simulink model "azimuth_wiith_variable_gain"  (R2025b)
settings: Solver=VariableStepAuto  StartTime=0.0  StopTime=10.0  RelTol=1e-3
values from neighbouring files (symbols this model uses):
  Kfar = 300    [nl_gain_demo.m]    (also in pVsScheduledPd.m)
  Knear = 60    [nl_gain_demo.m]    (also in pVsScheduledPd.m)
libraries: fl_lib x86, nesl_utility x15, simulink x2
settings Model: Creator=Lenovo  LastModifiedBy=Lenovo

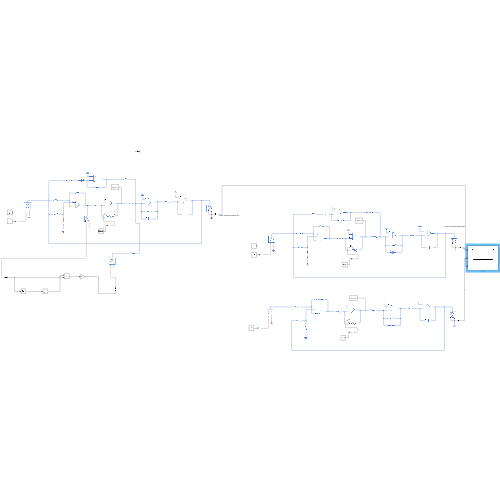
[thumbnail: Simulink's stored preview of the top-level diagram]
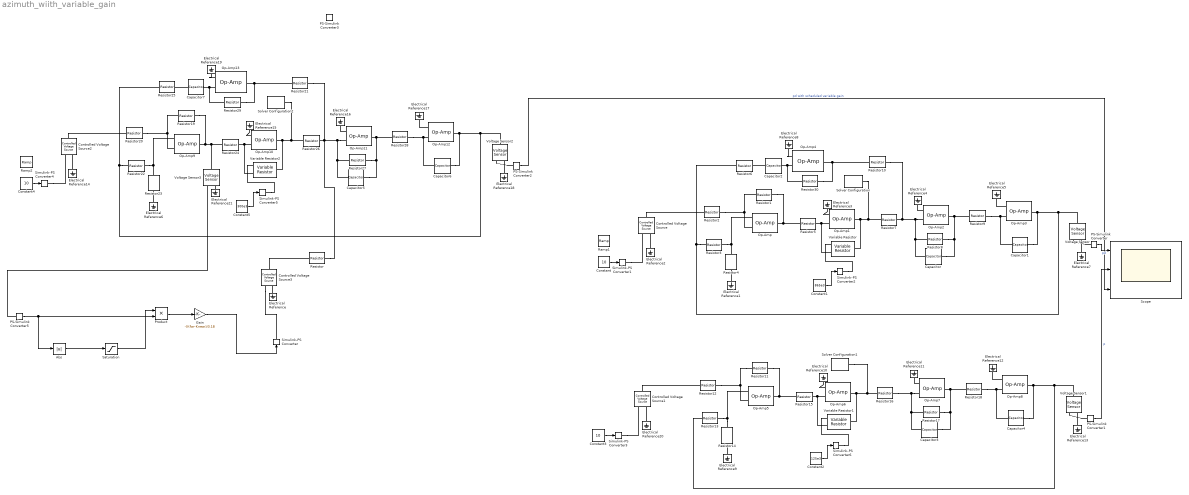
== system azimuth_wiith_variable_gain ==
  Abs : Abs  SaturateOnIntegerOverflow=off
  Capacitor{,1..7} (8 alike) : fl_lib/Electrical/Electrical Elements/Capacitor  c=1e-6 F  r=1e-6 Ohm  g=0 1/Ohm  i_specify=off  i_priority=None  i=0 A  i_nominal_specify=off  i_nominal_value=1  i_nominal_unit=A  v_specify=off  v_priority=None  v=0 V  v_nominal_specify=off  v_nominal_value=1  v_nominal_unit=V  vc_specify=off  vc_priority=High  vc=0 V  vc_nominal_specify=off  vc_nominal_value=1  vc_nominal_unit=V
  Constant : Constant  Value=10
  Constant1 : Constant  Value=865e3
  Constant2 : Constant  Value=125e3
  Constant3 : Constant  Value=10
  Constant4 : Constant  Value=10
  Constant5 : Constant  Value=300e3
  Controlled Voltage Source{,1..3} (4 alike) : fl_lib/Electrical/Electrical Sources/Controlled Voltage Source
  Electrical Reference{,1..21} (22 alike) : fl_lib/Electrical/Electrical Elements/Electrical Reference
  Gain : Gain  Gain=-(Kfar-Knear)/3.18
  Op-Amp{,1..13} (14 alike) : fl_lib/Electrical/Electrical Elements/Op-Amp  outI_specify=off  outI_priority=None  outI=0 A  outI_nominal_specify=off  outI_nominal_value=1  outI_nominal_unit=A
  PS-Simulink Converter{,1..3,5} (5 alike) : nesl_utility/PS-Simulink Converter  PhysicalDomain=network_engine_domain  SubClassName=ps_output  LeftPortType=input  RightPortType=output  PseudoPeriodic=off  Frequencies=[]  VectorFormat=inherit  Unit=inherit  AffineConversion=off
  Product : Product
  Ramp1 : simulink/Sources/Ramp  slope=1  start=0  InitialOutput=0
  Ramp2 : simulink/Sources/Ramp  slope=1  start=0  InitialOutput=0
  Resistor : fl_lib/Electrical/Electrical Elements/Resistor  R=4.87 MOhm  i_specify=off  i_priority=None  i=0 A  i_nominal_specify=off  i_nominal_value=1  i_nominal_unit=A  v_specify=off  v_priority=None  v=0 V  v_nominal_specify=off  v_nominal_value=1  v_nominal_unit=V
  Resistor{1,4,11,14,19,23} (6 alike) : fl_lib/Electrical/Electrical Elements/Resistor  R=31.8 kOhm  i_specify=off  i_priority=None  i=0 A  i_nominal_specify=off  i_nominal_value=1  i_nominal_unit=A  v_specify=off  v_priority=None  v=0 V  v_nominal_specify=off  v_nominal_value=1  v_nominal_unit=V
  Resistor10 : fl_lib/Electrical/Electrical Elements/Resistor  R=4.87 MOhm  i_specify=off  i_priority=None  i=0 A  i_nominal_specify=off  i_nominal_value=1  i_nominal_unit=A  v_specify=off  v_priority=None  v=0 V  v_nominal_specify=off  v_nominal_value=1  v_nominal_unit=V
  Resistor{2..3,12..13,20,22} (6 alike) : fl_lib/Electrical/Electrical Elements/Resistor  R=100 kOhm  i_specify=off  i_priority=None  i=0 A  i_nominal_specify=off  i_nominal_value=1  i_nominal_unit=A  v_specify=off  v_priority=None  v=0 V  v_nominal_specify=off  v_nominal_value=1  v_nominal_unit=V
  Resistor15 : fl_lib/Electrical/Electrical Elements/Resistor  R=5 kOhm  i_specify=off  i_priority=None  i=0 A  i_nominal_specify=off  i_nominal_value=1  i_nominal_unit=A  v_specify=off  v_priority=None  v=0 V  v_nominal_specify=off  v_nominal_value=1  v_nominal_unit=V
  Resistor16 : fl_lib/Electrical/Electrical Elements/Resistor  R=4.8 MOhm  i_specify=off  i_priority=None  i=0 A  i_nominal_specify=off  i_nominal_value=1  i_nominal_unit=A  v_specify=off  v_priority=None  v=0 V  v_nominal_specify=off  v_nominal_value=1  v_nominal_unit=V
  Resistor17 : fl_lib/Electrical/Electrical Elements/Resistor  R=585 kOhm  i_specify=off  i_priority=None  i=0 A  i_nominal_specify=off  i_nominal_value=1  i_nominal_unit=A  v_specify=off  v_priority=None  v=0 V  v_nominal_specify=off  v_nominal_value=1  v_nominal_unit=V
  Resistor18 : fl_lib/Electrical/Electrical Elements/Resistor  R=1 MOhm  i_specify=off  i_priority=None  i=0 A  i_nominal_specify=off  i_nominal_value=1  i_nominal_unit=A  v_specify=off  v_priority=None  v=0 V  v_nominal_specify=off  v_nominal_value=1  v_nominal_unit=V
  Resistor21 : fl_lib/Electrical/Electrical Elements/Resistor  R=4.87 MOhm  i_specify=off  i_priority=None  i=0 A  i_nominal_specify=off  i_nominal_value=1  i_nominal_unit=A  v_specify=off  v_priority=None  v=0 V  v_nominal_specify=off  v_nominal_value=1  v_nominal_unit=V
  Resistor24 : fl_lib/Electrical/Electrical Elements/Resistor  R=5 kOhm  i_specify=off  i_priority=None  i=0 A  i_nominal_specify=off  i_nominal_value=1  i_nominal_unit=A  v_specify=off  v_priority=None  v=0 V  v_nominal_specify=off  v_nominal_value=1  v_nominal_unit=V
  Resistor25 : fl_lib/Electrical/Electrical Elements/Resistor  R=10 kOhm  i_specify=off  i_priority=None  i=0 A  i_nominal_specify=off  i_nominal_value=1  i_nominal_unit=A  v_specify=off  v_priority=None  v=0 V  v_nominal_specify=off  v_nominal_value=1  v_nominal_unit=V
  Resistor26 : fl_lib/Electrical/Electrical Elements/Resistor  R=4.8 MOhm  i_specify=off  i_priority=None  i=0 A  i_nominal_specify=off  i_nominal_value=1  i_nominal_unit=A  v_specify=off  v_priority=None  v=0 V  v_nominal_specify=off  v_nominal_value=1  v_nominal_unit=V
  Resistor27 : fl_lib/Electrical/Electrical Elements/Resistor  R=585 kOhm  i_specify=off  i_priority=None  i=0 A  i_nominal_specify=off  i_nominal_value=1  i_nominal_unit=A  v_specify=off  v_priority=None  v=0 V  v_nominal_specify=off  v_nominal_value=1  v_nominal_unit=V
  Resistor28 : fl_lib/Electrical/Electrical Elements/Resistor  R=1 MOhm  i_specify=off  i_priority=None  i=0 A  i_nominal_specify=off  i_nominal_value=1  i_nominal_unit=A  v_specify=off  v_priority=None  v=0 V  v_nominal_specify=off  v_nominal_value=1  v_nominal_unit=V
  Resistor29 : fl_lib/Electrical/Electrical Elements/Resistor  R=15 MOhm  i_specify=off  i_priority=None  i=0 A  i_nominal_specify=off  i_nominal_value=1  i_nominal_unit=A  v_specify=off  v_priority=None  v=0 V  v_nominal_specify=off  v_nominal_value=1  v_nominal_unit=V
  Resistor30 : fl_lib/Electrical/Electrical Elements/Resistor  R=11 MOhm  i_specify=off  i_priority=None  i=0 A  i_nominal_specify=off  i_nominal_value=1  i_nominal_unit=A  v_specify=off  v_priority=None  v=0 V  v_nominal_specify=off  v_nominal_value=1  v_nominal_unit=V
  Resistor5 : fl_lib/Electrical/Electrical Elements/Resistor  R=5 kOhm  i_specify=off  i_priority=None  i=0 A  i_nominal_specify=off  i_nominal_value=1  i_nominal_unit=A  v_specify=off  v_priority=None  v=0 V  v_nominal_specify=off  v_nominal_value=1  v_nominal_unit=V
  Resistor6 : fl_lib/Electrical/Electrical Elements/Resistor  R=10 kOhm  i_specify=off  i_priority=None  i=0 A  i_nominal_specify=off  i_nominal_value=1  i_nominal_unit=A  v_specify=off  v_priority=None  v=0 V  v_nominal_specify=off  v_nominal_value=1  v_nominal_unit=V
  Resistor7 : fl_lib/Electrical/Electrical Elements/Resistor  R=4.8 MOhm  i_specify=off  i_priority=None  i=0 A  i_nominal_specify=off  i_nominal_value=1  i_nominal_unit=A  v_specify=off  v_priority=None  v=0 V  v_nominal_specify=off  v_nominal_value=1  v_nominal_unit=V
  Resistor8 : fl_lib/Electrical/Electrical Elements/Resistor  R=585 kOhm  i_specify=off  i_priority=None  i=0 A  i_nominal_specify=off  i_nominal_value=1  i_nominal_unit=A  v_specify=off  v_priority=None  v=0 V  v_nominal_specify=off  v_nominal_value=1  v_nominal_unit=V
  Resistor9 : fl_lib/Electrical/Electrical Elements/Resistor  R=1 MOhm  i_specify=off  i_priority=None  i=0 A  i_nominal_specify=off  i_nominal_value=1  i_nominal_unit=A  v_specify=off  v_priority=None  v=0 V  v_nominal_specify=off  v_nominal_value=1  v_nominal_unit=V
  Saturation : Saturate  UpperLimit=3.18  LowerLimit=0
  Scope : Scope  NumInputPorts=3
      settings: ActiveDisplayYMinimum=-9.3038927314256714  ActiveDisplayYMaximum=26.895222046777043
  Simulink-PS Converter{,1..6} (7 alike) : nesl_utility/Simulink-PS Converter  PhysicalDomain=network_engine_domain  SubClassName=ps_input  LeftPortType=input  RightPortType=output  PseudoPeriodic=off  Frequencies=[]  NoiseDistribution=none  NoiseParameters=[]  Unit=1  AffineConversion=off  FilteringAndDerivatives=provide  SimscapeFilterOrder=1  InputFilterTimeConstant=0.001  UdotUserProvided=0
  Solver Configuration : nesl_utility/Solver Configuration  PhysicalDomain=network_engine_domain  SubClassName=solver  LeftPortType=input  RightPortType=generic  Tones=[]  Harmonics=[]  SimulateNoise=off  Profile=off  UseLocalSampling=off  EnableSwitchedLinearOptims=on  FrequencyDomain=off  UseCCode=off  RelTol=0.001  AbsTol=0.001  MinStep=1e-09  ToWorkspace=off  RevertToSquareIcSolve=off  NumHomotopyIterations=100  PhasorMode=off  PhasorModeNumHarmonics=1  ConsistencySolver=NEWTON_XTOL_AFTER_FTOL  IndexReductionMethod=DerivativeReplacement  DoDC=off  ResidualTolerance=1e-09  ConsistencyTolSource=GLOBAL  ConsistencyAbsTol=0.001  ConsistencyRelTol=0.001  ConsistencyTolFactor=0.001  UseLocalSolver=off  LocalSolverChoice=NE_BACKWARD_EULER_ADVANCER  ResolveIndetEquations=on  FunctionEvalNumThread=1  LocalSolverSampleTime=0.001  DoFixedCost=off  MaxNonlinIter=3  MaxModeIter=2  ComputeImpulses=off  ImpulseIterations=2  LinearAlgebra=auto  LinearAlgebraNumThread=0  EquationFormulation=NE_TIME_EF  DelaysMemoryBudget=1024  AutomaticFiltering=on  FilteringTimeConstant=0.001  PartitionStorageMethod=AS_NEEDED  PartitionMemoryBudget=1024  PartitionMethod=ROBUST  MultibodyUseLocalSolver=off  MultibodyLocalSolverChoice=ODE1  MultibodyLocalSolverSampleTime=0.001
  Solver Configuration1 : nesl_utility/Solver Configuration  PhysicalDomain=network_engine_domain  SubClassName=solver  LeftPortType=input  RightPortType=generic  Tones=[]  Harmonics=[]  SimulateNoise=off  Profile=off  UseLocalSampling=off  EnableSwitchedLinearOptims=on  FrequencyDomain=off  UseCCode=off  RelTol=0.001  AbsTol=0.001  MinStep=1e-09  ToWorkspace=off  RevertToSquareIcSolve=off  NumHomotopyIterations=100  PhasorMode=off  PhasorModeNumHarmonics=1  ConsistencySolver=NEWTON_XTOL_AFTER_FTOL  IndexReductionMethod=DerivativeReplacement  DoDC=off  ResidualTolerance=1e-09  ConsistencyTolSource=GLOBAL  ConsistencyAbsTol=0.001  ConsistencyRelTol=0.001  ConsistencyTolFactor=0.001  UseLocalSolver=off  LocalSolverChoice=NE_BACKWARD_EULER_ADVANCER  ResolveIndetEquations=on  FunctionEvalNumThread=1  LocalSolverSampleTime=0.001  DoFixedCost=off  MaxNonlinIter=3  MaxModeIter=2  ComputeImpulses=off  ImpulseIterations=2  LinearAlgebra=auto  LinearAlgebraNumThread=0  EquationFormulation=NE_TIME_EF  DelaysMemoryBudget=1024  AutomaticFiltering=on  FilteringTimeConstant=0.001  PartitionStorageMethod=AS_NEEDED  PartitionMemoryBudget=1024  PartitionMethod=ROBUST  MultibodyUseLocalSolver=off  MultibodyLocalSolverChoice=ODE1  MultibodyLocalSolverSampleTime=0.001
  Solver Configuration2 : nesl_utility/Solver Configuration  PhysicalDomain=network_engine_domain  SubClassName=solver  LeftPortType=input  RightPortType=generic  Tones=[]  Harmonics=[]  SimulateNoise=off  Profile=off  UseLocalSampling=off  EnableSwitchedLinearOptims=on  FrequencyDomain=off  UseCCode=off  RelTol=0.001  AbsTol=0.001  MinStep=1e-09  ToWorkspace=off  RevertToSquareIcSolve=off  NumHomotopyIterations=100  PhasorMode=off  PhasorModeNumHarmonics=1  ConsistencySolver=NEWTON_XTOL_AFTER_FTOL  IndexReductionMethod=DerivativeReplacement  DoDC=off  ResidualTolerance=1e-09  ConsistencyTolSource=GLOBAL  ConsistencyAbsTol=0.001  ConsistencyRelTol=0.001  ConsistencyTolFactor=0.001  UseLocalSolver=off  LocalSolverChoice=NE_BACKWARD_EULER_ADVANCER  ResolveIndetEquations=on  FunctionEvalNumThread=1  LocalSolverSampleTime=0.001  DoFixedCost=off  MaxNonlinIter=3  MaxModeIter=2  ComputeImpulses=off  ImpulseIterations=2  LinearAlgebra=auto  LinearAlgebraNumThread=0  EquationFormulation=NE_TIME_EF  DelaysMemoryBudget=1024  AutomaticFiltering=on  FilteringTimeConstant=0.001  PartitionStorageMethod=AS_NEEDED  PartitionMemoryBudget=1024  PartitionMethod=ROBUST  MultibodyUseLocalSolver=off  MultibodyLocalSolverChoice=ODE1  MultibodyLocalSolverSampleTime=0.001
  Variable Resistor : fl_lib/Electrical/Electrical Elements/Variable Resistor  Rmin=0 Ohm  thermalEnable=false  thermal_mass=1 J/K  i_specify=off  i_priority=None  i=0 A  i_nominal_specify=off  i_nominal_value=1  i_nominal_unit=A  v_specify=off  v_priority=None  v=0 V  v_nominal_specify=off  v_nominal_value=1  v_nominal_unit=V  T_specify=off  T_priority=None  T=300 K  T_nominal_specify=off  T_nominal_value=1  T_nominal_unit=K
  Variable Resistor1 : fl_lib/Electrical/Electrical Elements/Variable Resistor  Rmin=0 Ohm  thermalEnable=false  thermal_mass=1 J/K  i_specify=off  i_priority=None  i=0 A  i_nominal_specify=off  i_nominal_value=1  i_nominal_unit=A  v_specify=off  v_priority=None  v=0 V  v_nominal_specify=off  v_nominal_value=1  v_nominal_unit=V  T_specify=off  T_priority=None  T=300 K  T_nominal_specify=off  T_nominal_value=1  T_nominal_unit=K
  Variable Resistor2 : fl_lib/Electrical/Electrical Elements/Variable Resistor  Rmin=0 Ohm  thermalEnable=false  thermal_mass=1 J/K  i_specify=off  i_priority=None  i=0 A  i_nominal_specify=off  i_nominal_value=1  i_nominal_unit=A  v_specify=off  v_priority=None  v=0 V  v_nominal_specify=off  v_nominal_value=1  v_nominal_unit=V  T_specify=off  T_priority=None  T=300 K  T_nominal_specify=off  T_nominal_value=1  T_nominal_unit=K
  Voltage Sensor{,1..3} (4 alike) : fl_lib/Electrical/Electrical Sensors/Voltage Sensor
  wires:
  Constant4/1 -> Simulink-PS Converter4/1
  Constant5/1 -> Simulink-PS Converter5/1
  PS-Simulink Converter2/1 -> Scope/3  "pd with scheduled variable gain"
  Product/1 -> Gain/1
  Abs/1 -> Saturation/1
  Saturation/1 -> Product/1
  Gain/1 -> Simulink-PS Converter/1
  PS-Simulink Converter/1 -> Scope/1  "pd"
  Constant/1 -> Simulink-PS Converter1/1
  Constant3/1 -> Simulink-PS Converter3/1
  Constant1/1 -> Simulink-PS Converter2/1
  PS-Simulink Converter1/1 -> Scope/2  "p"
  Constant2/1 -> Simulink-PS Converter6/1
  PS-Simulink Converter5/1 -> Abs/1, Product/2
  connections:
  Resistor24/RConn1 -- Op-Amp10/LConn2 -- Variable Resistor2/LConn2
  Resistor27/RConn1 -- Capacitor5/RConn1 -- Resistor28/LConn1 -- Op-Amp11/RConn1
  Op-Amp12/LConn2 -- Resistor28/RConn1 -- Capacitor6/LConn1
  Resistor22/LConn1 -- Resistor25/LConn1 -- Voltage Sensor2/LConn1 -- Op-Amp12/RConn1 -- Capacitor6/RConn1
  Solver Configuration2/RConn1 -- Resistor26/LConn1 -- Variable Resistor2/RConn1 -- Op-Amp10/RConn1
  Op-Amp9/RConn1 -- Resistor24/LConn1 -- Voltage Sensor3/LConn1 -- Resistor19/RConn1
  Op-Amp13/RConn1 -- Resistor21/LConn1 -- Resistor29/RConn1
  Op-Amp9/LConn2 -- Resistor20/RConn1 -- Resistor19/LConn1
  Op-Amp11/LConn2 -- Capacitor5/LConn1 -- Resistor27/LConn1 -- Resistor/RConn1 -- Resistor26/RConn1 -- Resistor21/RConn1
  Op-Amp13/LConn2 -- Capacitor7/RConn1 -- Resistor29/LConn1
  Op-Amp9/LConn1 -- Resistor22/RConn1 -- Resistor23/LConn1
  Electrical Reference6/LConn1 -- Resistor23/RConn1
  Electrical Reference14/LConn1 -- Controlled Voltage Source2/RConn2
  Simulink-PS Converter5/RConn1 -- Variable Resistor2/LConn1
  Simulink-PS Converter4/RConn1 -- Controlled Voltage Source2/RConn1
  Op-Amp11/LConn1 -- Electrical Reference16/LConn1
  PS-Simulink Converter2/LConn1 -- Voltage Sensor2/RConn1
  Op-Amp12/LConn1 -- Electrical Reference17/LConn1
  Op-Amp10/LConn1 -- Electrical Reference15/LConn1
  Capacitor7/LConn1 -- Resistor25/RConn1
  Op-Amp13/LConn1 -- Electrical Reference19/LConn1
  Electrical Reference18/LConn1 -- Voltage Sensor2/RConn2
  Controlled Voltage Source2/LConn1 -- Resistor20/LConn1
  Controlled Voltage Source3/RConn1 -- Simulink-PS Converter/RConn1
  Electrical Reference/LConn1 -- Controlled Voltage Source3/RConn2
  Controlled Voltage Source3/LConn1 -- Resistor/LConn1
  Op-Amp1/RConn1 -- Variable Resistor/RConn1 -- Resistor7/LConn1 -- Solver Configuration/RConn1
  Variable Resistor1/LConn2 -- Resistor15/RConn1 -- Op-Amp6/LConn2
  Resistor16/LConn1 -- Op-Amp6/RConn1 -- Variable Resistor1/RConn1 -- Solver Configuration1/RConn1
  Op-Amp2/LConn2 -- Capacitor/LConn1 -- Resistor8/LConn1 -- Resistor7/RConn1 -- Resistor10/RConn1
  Capacitor4/RConn1 -- Voltage Sensor1/LConn1 -- Resistor13/LConn1 -- Op-Amp8/RConn1
  Op-Amp4/LConn2 -- Capacitor2/RConn1 -- Resistor30/LConn1
  Capacitor4/LConn1 -- Op-Amp8/LConn2 -- Resistor18/RConn1
  Resistor11/RConn1 -- Op-Amp5/RConn1 -- Resistor15/LConn1
  Resistor11/LConn1 -- Op-Amp5/LConn2 -- Resistor12/RConn1
  Resistor17/RConn1 -- Capacitor3/RConn1 -- Op-Amp7/RConn1 -- Resistor18/LConn1
  Op-Amp/RConn1 -- Resistor5/LConn1 -- Resistor1/RConn1
  Op-Amp/LConn1 -- Resistor3/RConn1 -- Resistor4/LConn1
  Op-Amp4/RConn1 -- Resistor10/LConn1 -- Resistor30/RConn1
  Op-Amp7/LConn2 -- Resistor17/LConn1 -- Capacitor3/LConn1 -- Resistor16/RConn1
  Resistor8/RConn1 -- Resistor9/LConn1 -- Op-Amp2/RConn1 -- Capacitor/RConn1
  Resistor3/LConn1 -- Resistor6/LConn1 -- Op-Amp3/RConn1 -- Capacitor1/RConn1 -- Voltage Sensor/LConn1
  Resistor14/LConn1 -- Op-Amp5/LConn1 -- Resistor13/RConn1
  Op-Amp/LConn2 -- Resistor2/RConn1 -- Resistor1/LConn1
  Resistor5/RConn1 -- Op-Amp1/LConn2 -- Variable Resistor/LConn2
  Op-Amp3/LConn2 -- Resistor9/RConn1 -- Capacitor1/LConn1
  Simulink-PS Converter3/RConn1 -- Controlled Voltage Source1/RConn1
  Op-Amp4/LConn1 -- Electrical Reference8/LConn1
  Op-Amp7/LConn1 -- Electrical Reference11/LConn1
  Electrical Reference7/LConn1 -- Voltage Sensor/RConn2
  Electrical Reference13/LConn1 -- Voltage Sensor1/RConn2
  Electrical Reference9/LConn1 -- Resistor14/RConn1
  PS-Simulink Converter/LConn1 -- Voltage Sensor/RConn1
  Op-Amp8/LConn1 -- Electrical Reference12/LConn1
  Op-Amp1/LConn1 -- Electrical Reference3/LConn1
  Op-Amp3/LConn1 -- Electrical Reference5/LConn1
  Op-Amp6/LConn1 -- Electrical Reference10/LConn1
  Simulink-PS Converter2/RConn1 -- Variable Resistor/LConn1
  Electrical Reference20/LConn1 -- Controlled Voltage Source1/RConn2
  Controlled Voltage Source/LConn1 -- Resistor2/LConn1
  Capacitor2/LConn1 -- Resistor6/RConn1
  Op-Amp2/LConn1 -- Electrical Reference4/LConn1
  PS-Simulink Converter1/LConn1 -- Voltage Sensor1/RConn1
  Controlled Voltage Source1/LConn1 -- Resistor12/LConn1
  Electrical Reference1/LConn1 -- Resistor4/RConn1
  Simulink-PS Converter1/RConn1 -- Controlled Voltage Source/RConn1
  Simulink-PS Converter6/RConn1 -- Variable Resistor1/LConn1
  Electrical Reference2/LConn1 -- Controlled Voltage Source/RConn2
  Electrical Reference21/LConn1 -- Voltage Sensor3/RConn2
  PS-Simulink Converter5/LConn1 -- Voltage Sensor3/RConn1
